simulink model "QD2_DroneStack_MPC"  (R2023a)
settings: Solver=ode1  StartTime=0.0  StopTime=inf  FixedStep=1/1000  RelTol=1e-3  EnableMultiTasking=on
InitFcn:
  | % QD2_DroneStack_MPC: rutas de la librería qd2_* y del mapeo de motores
  | qd2_d = fileparts(get_param(bdroot, 'FileName'));
  | for qd2_k = 1:4
  |     if exist(fullfile(qd2_d, 'lib', 'qd2_params.m'), 'file'), break; end
  |     qd2_d = fileparts(qd2_d);
  | end
  | addpath(fullfile(qd2_d, 'lib'));
  | addpath(fullfile(qd2_d, 'equipo2_original'));
  | clear qd2_d qd2_k
  | Motor_Mapping_7_Inch
model workspace (MAT data in the model file):
  target_system = 1
undefined symbols (not defined in the file): _Commander, _QDrone2, _Stabilizer, datetime, HIL, KT, lf, log_, m, Motor_Matrix, n, qc_get_step_size, s, saved_data
libraries: quarc_library x94, simulink x27, simulink_extras x9
(part 4 of 5)

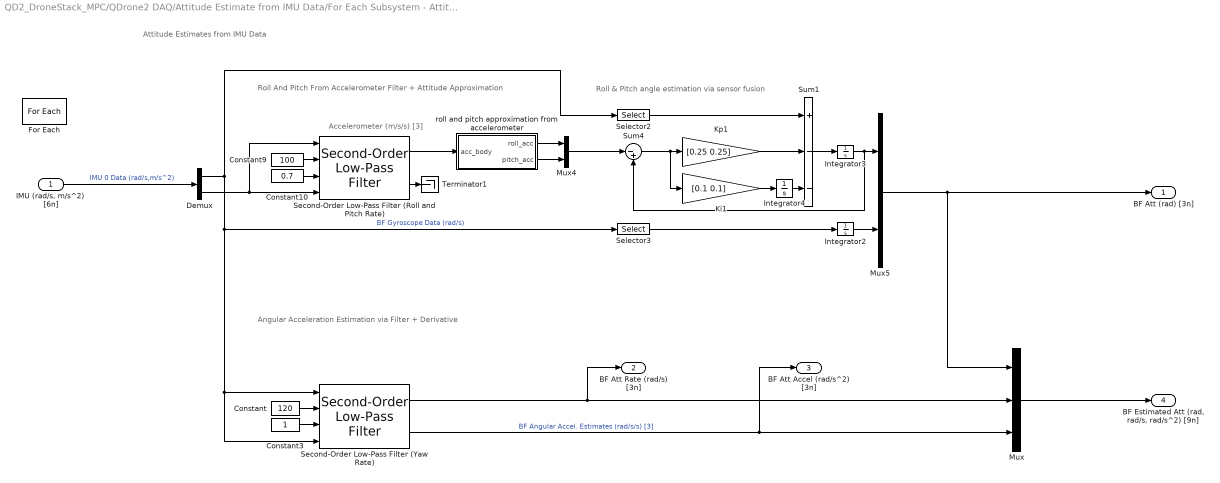
== system QD2_DroneStack_MPC/QDrone2 DAQ/Attitude Estimate from IMU Data/For Each Subsystem - Attitutde Estimates ==
  note: Attitude Estimates from IMU Data
  note: Accelerometer (m/s/s) [3]
  note: Roll And Pitch From Accelerometer Filter + Attitude Approximation
  note: Roll & Pitch angle estimation via sensor fusion
  note: Angular Acceleration Estimation via Filter + Derivative
  "IMU (rad/s, m/s^2) [6n]" : Inport  Partition=on  PartitionDimension=1  PartitionWidth=6  PartitionOffset=0
  Constant : Constant  Value=120
  Constant10 : Constant  Value=0.7
  Constant3 : Constant
  Constant9 : Constant  Value=100
  Demux : Demux  Outputs=[3,3]
  For Each : ForEach  DisableCoverage=on
  Integrator2 : Integrator
  Integrator3 : Integrator
  Integrator4 : Integrator
  Ki1 : Gain  Gain=[0.1 0.1]
  Kp1 : Gain  Gain=[0.25 0.25]
  Mux : Mux  Inputs=3
  Mux4 : Mux  Inputs=2
  Mux5 : Mux  Inputs=2
  Second-Order Low-Pass Filter (Roll and Pitch Rate) : quarc_library/Continuous/Second-Order Low-Pass Filter  params_source=External (input ports)  input_width=200  input_zeta=1  input_init=0
  Second-Order Low-Pass Filter (Yaw Rate) : quarc_library/Continuous/Second-Order Low-Pass Filter  params_source=External (input ports)  input_width=200  input_zeta=1  input_init=0
  Selector2 : Selector  InputPortWidth=3  IndexOptions=Index vector (dialog)  Indices=[1,2]  OutputSizes=1
  Selector3 : Selector  InputPortWidth=3  IndexOptions=Index vector (dialog)  Indices=[3]  OutputSizes=1
  Sum1 : Sum  Inputs=+--
  Sum4 : Sum  Inputs=|-+
  Terminator1 : Terminator
  roll and pitch approximation from accelerometer : MATLAB Function  TreatAsAtomicUnit=on
  BF Att (rad) [3n] : Outport  ConcatenationDimension=1
  BF Att Rate (rad/s) [3n] : Outport  Port=2  ConcatenationDimension=1
  BF Att Accel (rad/s^2) [3n] : Outport  Port=3  ConcatenationDimension=1
  "BF Estimated Att (rad, rad/s, rad/s^2) [9n] " : Outport  Port=4  ConcatenationDimension=1
  wires:
  roll and pitch approximation from accelerometer/2(pitch_acc) -> Mux4/2
  Constant9/1 -> Second-Order Low-Pass Filter (Roll and Pitch Rate)/2
  Second-Order Low-Pass Filter (Roll and Pitch Rate)/1 -> roll and pitch approximation from accelerometer/1(acc_body)
  "IMU (rad/s, m/s^2) [6n]"/1 -> Demux/1  "IMU 0 Data (rad/s,m/s^2)"
  Constant10/1 -> Second-Order Low-Pass Filter (Roll and Pitch Rate)/3
  Demux/2 -> Second-Order Low-Pass Filter (Roll and Pitch Rate)/4, Second-Order Low-Pass Filter (Roll and Pitch Rate)/1
  Second-Order Low-Pass Filter (Roll and Pitch Rate)/2 -> Terminator1/1
  Selector3/1 -> Integrator2/1
  Integrator2/1 -> Mux5/2
  Integrator4/1 -> Sum1/3
  Kp1/1 -> Sum1/2
  Selector2/1 -> Sum1/1
  Integrator3/1 -> Sum4/2, Mux5/1
  Mux5/1 -> BF Att (rad) [3n]/1, Mux/1
  Sum4/1 -> Ki1/1, Kp1/1
  Sum1/1 -> Integrator3/1
  Ki1/1 -> Integrator4/1
  roll and pitch approximation from accelerometer/1(roll_acc) -> Mux4/1
  Mux4/1 -> Sum4/1
  Constant3/1 -> Second-Order Low-Pass Filter (Yaw Rate)/3
  Demux/1 -> Second-Order Low-Pass Filter (Yaw Rate)/4, Second-Order Low-Pass Filter (Yaw Rate)/1, Selector3/1, Selector2/1  "BF Gyroscope Data (rad/s)"
  Constant/1 -> Second-Order Low-Pass Filter (Yaw Rate)/2
  Second-Order Low-Pass Filter (Yaw Rate)/1 -> Mux/2, BF Att Rate (rad/s) [3n]/1
  Second-Order Low-Pass Filter (Yaw Rate)/2 -> BF Att Accel (rad/s^2) [3n]/1, Mux/3  "BF Angular Accel. Estimates (rad/s/s) [3]"
  Mux/1 -> "BF Estimated Att (rad, rad/s, rad/s^2) [9n] "/1

== system QD2_DroneStack_MPC/QDrone2 DAQ/Check Battery level/Triggered Subsystem ==
  Trigger : TriggerPort  VariantControl=(inherit)
  Constant : Constant
  Out1 : Outport  InitialOutput=[0]
  wires:
  Constant/1 -> Out1/1

== system QD2_DroneStack_MPC/QDrone2 DAQ/Sensor Failure Monitoring - IMU0/Sensor Failure (Accelerometer) ==
  note: Check for flat-line ZERO Accelerometer data (no data)
  Sensor Input : Inport
  Clock : Clock
  Compare To Constant : simulink/Logic and Bit Operations/Compare To Constant  relop=>=  const=1  OutDataTypeStr=boolean
  Demux1 : Demux  Outputs=3
  Logical Operator : Logic  Operator=OR  Inputs=3  AllPortsSameDT=off  OutDataTypeStr=boolean
  Logical Operator1 : Logic  AllPortsSameDT=off  OutDataTypeStr=boolean
  Terminator1 : Terminator
  Terminator3 : Terminator
  Terminator4 : Terminator
  Threshold : quarc_library/Discontinuities/Threshold  operator===  param_src=Specify via dialog  threshold=0  duration=1
      settings: SourceProductName=QUARC Targets
  Threshold1 : quarc_library/Discontinuities/Threshold  operator===  param_src=Specify via dialog  threshold=0  duration=1
      settings: SourceProductName=QUARC Targets
  Threshold2 : quarc_library/Discontinuities/Threshold  operator===  param_src=Specify via dialog  threshold=0  duration=1
      settings: SourceProductName=QUARC Targets
  Sensor Fault : Outport  VectorParamsAs1DForOutWhenUnconnected=off
  wires:
  Clock/1 -> Compare To Constant/1
  Threshold/1 -> Logical Operator/1
  Threshold1/1 -> Logical Operator/2
  Compare To Constant/1 -> Logical Operator1/1
  Logical Operator1/1 -> Sensor Fault/1
  Sensor Input/1 -> Demux1/1
  Threshold2/2 -> Terminator4/1
  Threshold2/1 -> Logical Operator/3
  Demux1/1 -> Threshold/1
  Demux1/3 -> Threshold2/1
  Demux1/2 -> Threshold1/1
  Logical Operator/1 -> Logical Operator1/2
  Threshold1/2 -> Terminator3/1
  Threshold/2 -> Terminator1/1

== system QD2_DroneStack_MPC/QDrone2 DAQ/Sensor Failure Monitoring - IMU0/Sensor Failure (Gyroscope) ==
  note: Check for flat-line ZERO Gyro data (no data)
  Sensor Input : Inport
  Clock : Clock
  Compare To Constant : simulink/Logic and Bit Operations/Compare To Constant  relop=>=  const=1  OutDataTypeStr=boolean
  Demux1 : Demux  Outputs=3
  Logical Operator : Logic  Operator=OR  Inputs=3  AllPortsSameDT=off  OutDataTypeStr=boolean
  Logical Operator1 : Logic  AllPortsSameDT=off  OutDataTypeStr=boolean
  Terminator1 : Terminator
  Terminator3 : Terminator
  Terminator4 : Terminator
  Threshold : quarc_library/Discontinuities/Threshold  operator===  param_src=Specify via dialog  threshold=0  duration=1
      settings: SourceProductName=QUARC Targets
  Threshold1 : quarc_library/Discontinuities/Threshold  operator===  param_src=Specify via dialog  threshold=0  duration=1
      settings: SourceProductName=QUARC Targets
  Threshold2 : quarc_library/Discontinuities/Threshold  operator===  param_src=Specify via dialog  threshold=0  duration=1
      settings: SourceProductName=QUARC Targets
  Sensor Fault : Outport  VectorParamsAs1DForOutWhenUnconnected=off
  wires:
  Threshold/2 -> Terminator1/1
  Threshold1/2 -> Terminator3/1
  Logical Operator/1 -> Logical Operator1/2
  Demux1/2 -> Threshold1/1
  Demux1/3 -> Threshold2/1
  Demux1/1 -> Threshold/1
  Threshold2/1 -> Logical Operator/3
  Threshold2/2 -> Terminator4/1
  Sensor Input/1 -> Demux1/1
  Logical Operator1/1 -> Sensor Fault/1
  Compare To Constant/1 -> Logical Operator1/1
  Threshold1/1 -> Logical Operator/2
  Threshold/1 -> Logical Operator/1
  Clock/1 -> Compare To Constant/1

== system QD2_DroneStack_MPC/QDrone2 DAQ/Sensor Failure Monitoring - IMU1/Sensor Failure (Accelerometer) ==
  note: Check for flat-line ZERO Accelerometer data (no data)
  Sensor Input : Inport
  Clock : Clock
  Compare To Constant : simulink/Logic and Bit Operations/Compare To Constant  relop=>=  const=1  OutDataTypeStr=boolean
  Demux1 : Demux  Outputs=3
  Logical Operator : Logic  Operator=OR  Inputs=3  AllPortsSameDT=off  OutDataTypeStr=boolean
  Logical Operator1 : Logic  AllPortsSameDT=off  OutDataTypeStr=boolean
  Terminator1 : Terminator
  Terminator3 : Terminator
  Terminator4 : Terminator
  Threshold : quarc_library/Discontinuities/Threshold  operator===  param_src=Specify via dialog  threshold=0  duration=1
      settings: SourceProductName=QUARC Targets
  Threshold1 : quarc_library/Discontinuities/Threshold  operator===  param_src=Specify via dialog  threshold=0  duration=1
      settings: SourceProductName=QUARC Targets
  Threshold2 : quarc_library/Discontinuities/Threshold  operator===  param_src=Specify via dialog  threshold=0  duration=1
      settings: SourceProductName=QUARC Targets
  Sensor Fault : Outport  VectorParamsAs1DForOutWhenUnconnected=off
  wires:
  Threshold/2 -> Terminator1/1
  Threshold1/2 -> Terminator3/1
  Logical Operator/1 -> Logical Operator1/2
  Demux1/2 -> Threshold1/1
  Demux1/3 -> Threshold2/1
  Demux1/1 -> Threshold/1
  Threshold2/1 -> Logical Operator/3
  Threshold2/2 -> Terminator4/1
  Sensor Input/1 -> Demux1/1
  Logical Operator1/1 -> Sensor Fault/1
  Compare To Constant/1 -> Logical Operator1/1
  Threshold1/1 -> Logical Operator/2
  Threshold/1 -> Logical Operator/1
  Clock/1 -> Compare To Constant/1

== system QD2_DroneStack_MPC/QDrone2 DAQ/Sensor Failure Monitoring - IMU1/Sensor Failure (Gyroscope) ==
  note: Check for flat-line ZERO Gyro data (no data)
  Sensor Input : Inport
  Clock : Clock
  Compare To Constant : simulink/Logic and Bit Operations/Compare To Constant  relop=>=  const=1  OutDataTypeStr=boolean
  Demux1 : Demux  Outputs=3
  Logical Operator : Logic  Operator=OR  Inputs=3  AllPortsSameDT=off  OutDataTypeStr=boolean
  Logical Operator1 : Logic  AllPortsSameDT=off  OutDataTypeStr=boolean
  Terminator1 : Terminator
  Terminator3 : Terminator
  Terminator4 : Terminator
  Threshold : quarc_library/Discontinuities/Threshold  operator===  param_src=Specify via dialog  threshold=0  duration=1
      settings: SourceProductName=QUARC Targets
  Threshold1 : quarc_library/Discontinuities/Threshold  operator===  param_src=Specify via dialog  threshold=0  duration=1
      settings: SourceProductName=QUARC Targets
  Threshold2 : quarc_library/Discontinuities/Threshold  operator===  param_src=Specify via dialog  threshold=0  duration=1
      settings: SourceProductName=QUARC Targets
  Sensor Fault : Outport  VectorParamsAs1DForOutWhenUnconnected=off
  wires:
  Clock/1 -> Compare To Constant/1
  Threshold/1 -> Logical Operator/1
  Threshold1/1 -> Logical Operator/2
  Compare To Constant/1 -> Logical Operator1/1
  Logical Operator1/1 -> Sensor Fault/1
  Sensor Input/1 -> Demux1/1
  Threshold2/2 -> Terminator4/1
  Threshold2/1 -> Logical Operator/3
  Demux1/1 -> Threshold/1
  Demux1/3 -> Threshold2/1
  Demux1/2 -> Threshold1/1
  Logical Operator/1 -> Logical Operator1/2
  Threshold1/2 -> Terminator3/1
  Threshold/2 -> Terminator1/1

== system QD2_DroneStack_MPC/QDrone2 DAQ/Subsystem1/Maintain previous value4 ==
  Value in : Inport
  Memory : Memory
  Switch : Switch  Criteria=u2 ~= 0  SaturateOnIntegerOverflow=off  InputSameDT=off
  Non 0 values : Outport
  wires:
  Value in/1 -> Switch/1, Switch/2
  Switch/1 -> Memory/1, Non 0 values/1
  Memory/1 -> Switch/3

== system QD2_DroneStack_MPC/COMMANDER (ANGLE MODE)/STATE MACHINE SIGNALS/Generate Extra Messages for Console/Boolean Edge-Based Triggered Print ==
  Signal Enable : Inport  Partition=on  PartitionDimension=1  PartitionWidth=1  PartitionOffset=0
  Message : Inport  Port=2  Partition=on  PartitionDimension=2  PartitionWidth=1  PartitionOffset=0
  time (s) : Inport  Port=3
  For Each : ForEach  DisableCoverage=on
  Triggered Subsystem1 : Subsystem  TreatAsAtomicUnit=on
  Out1 : Outport  ConcatenationDimension=1
  wires:
  time (s)/1 -> Triggered Subsystem1/1(Time (s))
  Message/1 -> Triggered Subsystem1/2(Message)
  Signal Enable/1 -> Out1/1, Triggered Subsystem1/Trigger

== system QD2_DroneStack_MPC/COMMANDER (ANGLE MODE)/STATE MACHINE SIGNALS/Generate State Messages for Console/Triggered Subsystem ==
  Value : Inport
  Time (s) : Inport  Port=2
  Message : Inport  Port=3
  Trigger : TriggerPort  VariantControl=(inherit)
  Data Type Conversion : DataTypeConversion  OutDataTypeStr=uint8  SaturateOnIntegerOverflow=off  RndMeth=Floor
  Print : quarc_library/User Interface/Standard I//O/Print  format_string="[ %lf ] (s): State %u  => %s \\n"  max_code_units=512  optimization=Minimizing latency  sample_time=-1  active=off
      settings: SourceProductName=QUARC Targets
  Terminator : Terminator
  Terminator1 : Terminator
  wires:
  Time (s)/1 -> Print/1
  Message/1 -> Print/3
  Print/2 -> Terminator/1
  Print/1 -> Terminator1/1
  Value/1 -> Data Type Conversion/1
  Data Type Conversion/1 -> Print/2

== system QD2_DroneStack_MPC/COMMANDER (ANGLE MODE)/STATE MACHINE SIGNALS/Generate Warning Messages for Console/Boolean Value-Based Triggered Print ==
  Signal Enable : Inport  Partition=on  PartitionDimension=1  PartitionWidth=1  PartitionOffset=0
  Message : Inport  Port=2  Partition=on  PartitionDimension=2  PartitionWidth=1  PartitionOffset=0
  time (s) : Inport  Port=3
  For Each : ForEach  DisableCoverage=on
  Triggered Subsystem : Subsystem  TreatAsAtomicUnit=on
  Out1 : Outport  ConcatenationDimension=1
  wires:
  time (s)/1 -> Triggered Subsystem/1(Time (s))
  Message/1 -> Triggered Subsystem/2(Message)
  Signal Enable/1 -> Triggered Subsystem/Trigger, Out1/1

== system QD2_DroneStack_MPC/COMMANDER (ANGLE MODE)/STATE MACHINE SIGNALS/Generate Extra Messages for Console/Boolean Edge-Based Triggered Print/Triggered Subsystem1 ==
  Time (s) : Inport
  Message : Inport  Port=2
  Trigger : TriggerPort  TriggerType=falling  VariantControl=(inherit)
  Print : quarc_library/User Interface/Standard I//O/Print  format_string=[ %lf ] (s): %s !\n  max_code_units=512  optimization=Minimizing latency  sample_time=-1  active=off
      settings: SourceProductName=QUARC Targets
  Terminator : Terminator
  Terminator1 : Terminator
  wires:
  Time (s)/1 -> Print/1
  Message/1 -> Print/2
  Print/2 -> Terminator/1
  Print/1 -> Terminator1/1

== system QD2_DroneStack_MPC/COMMANDER (ANGLE MODE)/STATE MACHINE SIGNALS/Generate Warning Messages for Console/Boolean Value-Based Triggered Print/Triggered Subsystem ==
  Time (s) : Inport
  Message : Inport  Port=2
  Trigger : TriggerPort  VariantControl=(inherit)
  Print : quarc_library/User Interface/Standard I//O/Print  format_string=[ %lf ] (s): %s\n  max_code_units=512  optimization=Minimizing latency  sample_time=-1  active=off
      settings: SourceProductName=QUARC Targets
  Terminator : Terminator
  Terminator1 : Terminator
  wires:
  Print/1 -> Terminator1/1
  Print/2 -> Terminator/1
  Message/1 -> Print/2
  Time (s)/1 -> Print/1

== matlab function QD2_DroneStack_MPC/HORIZON FRAME CONVERSION AND ESTIMATION/Pose Switchbox/MATLAB Function2 ==
  data: sigmoid_type input; enable output; height_des input; slow_lim input; fast_lim input; height_cur input; height_vel input; height_ref output; max_height_vel output; max_height_accel output
function [enable, height_ref, max_height_vel, max_height_accel] = fcn(sigmoid_type, height_des, slow_lim, fast_lim, height_cur, height_vel)

% Note: Some of the cases below are identical. However, they are separated out 
% based on the states of the state machine for ease of modification in the future. 
% For example, states 4 and 5 are identical. However, if the user wants different 
% signmoid behaviour when taking off than when landing, these cases may not be the same. 

enable = 0;
height_ref = 0;
max_height_vel = 0;
max_height_accel = 0;

switch sigmoid_type
    case 1 % This is for the IDLE, ARM, E_ABORT, E_STOP and DISABLE states of the FSM
        enable = 0;
        height_ref = 0;
        max_height_vel = 0;
        max_height_accel = 0;

    case 2 % This is for the TAKEOFF THROTTLE state of the FSM
        enable = 0;
        height_ref = 0;
        max_height_vel = 0;
        max_height_accel = 0;

    case 3 % This is for the FLIGHT state of the FSM 
        enable = 1;
        height_ref = height_des;
        max_height_vel = fast_lim(1);
        max_height_accel = fast_lim(2);

    case 4 % This is for the TAKEOFF HEIGHT state of the FSM
        enable = 1;
        height_ref = height_des;
        if (height_vel < 0)||(abs(height_cur - height_des) <= 0.1)||(height_des <= height_cur)
            max_height_vel = fast_lim(1);
            max_height_accel = fast_lim(2);
        else    
            max_height_vel = slow_lim(1);
            max_height_accel = slow_lim(2);
        end
    case 5 % This is for the AUTOLAND state of the FSM
        enable = 1;
        height_ref = 0;
        if height_vel >= 0
            max_height_vel = fast_lim(1);
            max_height_accel = fast_lim(2);        
        else
            max_height_vel = slow_lim(1);
            max_height_accel = slow_lim(2);
        end
        
end

== matlab function QD2_DroneStack_MPC/HORIZON FRAME CONVERSION AND ESTIMATION/Pose Switchbox/MATLAB Function4 ==
  data: sigmoid_type input; enable output; yaw_des input; slow_lim input; fast_lim input; yaw_cur input; yaw_ref output; max_yaw_vel output; max_yaw_accel output; yaw_vel input
function [enable, yaw_ref, max_yaw_vel, max_yaw_accel] = fcn(sigmoid_type, yaw_des, slow_lim, fast_lim, yaw_cur, yaw_vel)

% Note: Some of the cases below are identical. However, they are separated out 
% based on the states of the state machine for ease of modification in the future. 
% For example, states 4 and 5 are identical. However, if the user wants different 
% signmoid behaviour when taking off than when landing, these cases may not be the same. 

enable = 0;
yaw_ref = 0;
max_yaw_vel = 0;
max_yaw_accel = 0;

switch sigmoid_type
    case 1 % This is for the IDLE, ARM, E_ABORT, E_STOP and DISABLE states of the FSM
        enable = 0;
        yaw_ref = 0;
        max_yaw_vel = 0;
        max_yaw_accel = 0;
    case 2 % This is for the TAKEOFF THROTTLE state of the FSM
        enable = 1;
        yaw_ref = yaw_des;
        max_yaw_vel = slow_lim(1);
        max_yaw_accel = slow_lim(2);  
    case 3 % This is for the FLIGHT state of the FSM 
        enable = 1;
        yaw_ref = yaw_des;
        max_yaw_vel = fast_lim(1);
        max_yaw_accel = fast_lim(2);
    case 4 % This is for the TAKEOFF HEIGHT state of the FSM
        enable = 1;
        yaw_ref = yaw_des;
        if (yaw_vel < 0)||(yaw_des < yaw_cur)||(abs(yaw_cur-yaw_des)<=0.2)
            max_yaw_vel = fast_lim(1);
            max_yaw_accel = fast_lim(2);
        else    
            max_yaw_vel = slow_lim(1);
            max_yaw_accel = slow_lim(2);
        end
    case 5 % This is for the AUTOLAND state of the FSM
        enable = 1;
        yaw_ref = yaw_des;
        if (yaw_vel >= 0)
            max_yaw_vel = fast_lim(1);
            max_yaw_accel = fast_lim(2);
        else    
            max_yaw_vel = slow_lim(1);
            max_yaw_accel = slow_lim(2);
        end
end

== matlab function QD2_DroneStack_MPC/HORIZON FRAME CONVERSION AND ESTIMATION/Pose Switchbox/Signmoid Type ==
  data: FSM_state input; sigmoid_type output
function sigmoid_type  = sigmoid_type_position(FSM_state)

% QDrone: Position Switchbox
%
% Switching between different sigmoid types based on 
% which state the FSM is in.
%
% v3.0 - 4th October, 2018
%
% INPUTS:
% -------
% FSM_state = current state of the FSM------------------------------------------------------- (#)         [1]
% 
% OUTPUTS:
% --------
% sigmoid_type = an integer whose state determines how the commands/measurements are transformed-- (#)         [1]

% Sigmoid_type = 1; This is for the IDLE, ARM, E_ABORT, E_STOP and DISABLE states of the FSM
% Sigmoid_type = 2; This is for the TAKEOFF THROTTLE state of the FSM
% Sigmoid_type = 3; This is for the FLIGHT state of the FSM
% Sigmoid_type = 4; This is for the TAKEOFF HEIGHT state of the FSM
% Sigmoid_type = 5; This is for the AUTOLAND state of the FSM

sigmoid_type = 0;

switch FSM_state
    case 1 % IDLE STATE
        sigmoid_type = 1;
    case 2 % ARM STATE
        sigmoid_type = 1;
    case 3 % TAKEOFF THROTTLE STATE
        sigmoid_type = 2;
    case 4 % TAKEOFF HEIGHT STATE
        sigmoid_type = 4;
    case 5 % FLIGHT STATE
        sigmoid_type = 3;
    case 6 % AUTOLAND STATE
        sigmoid_type = 5;
    case 7 % EMERGENCY STOP STATE
        sigmoid_type = 1;
    case 8 % EMERGENCY ABORT STATE
        sigmoid_type = 1;
    case 9 % DISABLE STATE
        sigmoid_type = 1;
end

== matlab function QD2_DroneStack_MPC/COMMANDER (ANGLE MODE)/THROTTLE SWITCHBOX /Hover Throttle Sigmoid Parameters ==
  data: sigmoid_type input; enable output; trim_throttle input; takeoff_lim input; land_lim input; throttle_vel input; throttle_ref output; max_throttle_vel output; max_throttle_accel output
function [enable, throttle_ref, max_throttle_vel, max_throttle_accel] = fcn(sigmoid_type, trim_throttle, takeoff_lim, land_lim, throttle_vel)

% Note: Some of the cases below are identical. However, they are separated out 
% based on the states of the state machine for ease of modification in the future. 
% For example, states 4 and 5 are identical. However, if the user wants different 
% signmoid behaviour when taking off than when landing, these cases may not be the same. 

enable = 0;
throttle_ref = 0;
max_throttle_vel = 0;
max_throttle_accel = 0;

switch sigmoid_type
    case 1 % sigmoid = 1 - Command 0 throttle
        % This is for the IDLE, ARM, E_ABORT, and DISABLE states of the FSM
        enable = 0;
        throttle_ref = 0;
        max_throttle_vel = 0;
        max_throttle_accel = 0;

    case 2 % sigmoid = 2 - Sigmoid throttle up from 0 to the trim value
        % This is for the TAKEOFF THROTTLE state of the FSM
        enable = 1;
        throttle_ref = trim_throttle;
        max_throttle_vel = takeoff_lim(1);
        max_throttle_accel = takeoff_lim(2);

    case 3 % sigmoid = 3 - Pass controller throttle straight through + trim value.
        % This is for the TAKEOFF HEIGHT and FLIGHT state of the FSM
        enable = 1;
        throttle_ref = trim_throttle;
        max_throttle_vel = takeoff_lim(1);
        max_throttle_accel = takeoff_lim(2);

    case 4 % sigmoid = 4 - Ignore controller throttle. Sigmoid it down to 0.
        % This is for the E_Landing state of the FSM
        enable = 1;
        throttle_ref = 0;
        if throttle_vel > 0
            max_throttle_vel = takeoff_lim(1);
            max_throttle_accel = takeoff_lim(2);
        else
            max_throttle_vel = land_lim(1);
            max_throttle_accel = land_lim(2);
        end
        
    case 5 % sigmoid = 5 - Pass controller throttle straight through + trim value.
        % This is for the AUTOLAND state of the FSM
        enable = 1;
        throttle_ref = trim_throttle;
        max_throttle_vel = takeoff_lim(1);
        max_throttle_accel = takeoff_lim(2);

end

== matlab function QD2_DroneStack_MPC/COMMANDER (ANGLE MODE)/STATE MACHINE LOGIC ==
  data: E_Abort output; isArm output; pt_ARM_to_TAKEOFF_THROTTLE output; pt_TAKE_OFF_HEIGHT_TO_AUTOLAND output; pt_FLIGHT_TO_AUTOLAND output; current_state input; initializing input; Tracking_Issue input; Communication_Issue input; low_battery input; trigger_1 input; trigger_2 input; E_abort input; joystick_issue input; net_throttle_at_trim input; net_throttle_close_to_zero input; ctrl_throttle_close_to_zero input; take_off_successful input; flying_too_low input; flying_too_high input; close_to_ground input; pt_TAKEOFF_THROTTLE_TO_TAKEOFF_HEIGHT output; pt_TAKE_OFF_HEIGHT_TO_FLIGHT output; pt_AUTOLAND_TO_DISABLE output; pt_EMERGENCY_STOP_TO_DISABLE output; pt_EMERGENCY_ABORT_TO_DISABLE output; Error output; stop_model output; sensor_failed input
function [E_Abort, isArm, pt_ARM_to_TAKEOFF_THROTTLE, pt_TAKE_OFF_HEIGHT_TO_AUTOLAND, pt_FLIGHT_TO_AUTOLAND, pt_TAKEOFF_THROTTLE_TO_TAKEOFF_HEIGHT, pt_TAKE_OFF_HEIGHT_TO_FLIGHT, pt_AUTOLAND_TO_DISABLE, pt_EMERGENCY_STOP_TO_DISABLE, pt_EMERGENCY_ABORT_TO_DISABLE, Error, stop_model]...
    = SM_logic(current_state, initializing, Tracking_Issue, Communication_Issue, low_battery, trigger_1, trigger_2, E_abort, joystick_issue,...
    net_throttle_at_trim, net_throttle_close_to_zero, ctrl_throttle_close_to_zero, take_off_successful, flying_too_low, flying_too_high, close_to_ground, sensor_failed)

% Programmatic Logic Block
%
% Logic for the FSM is generated here based on a variety of signals.
% Mostly, logic to programmatically trigger the transition to either a 
% natural next state, or an Error state, is generated here.
%
% Last modified: March, 2020
%
% INPUTS:
% -------
% current_state = previous state of the FSM-------------------------------------------------- (#)         [1]
% initializing = signal representing that the system is initializing (first 5s + buffer)- - - (bool)      [1]
% comm = communication signal representing MAVLINK connection-------------------------------- (bool)      [1]
% peripheral = signal representing joystick and optitrack connection- - - - - - - - - - - - - (bool)      [2]
% low_battery = signal representing low battery---------------------------------------------- (bool)      [1]
% trigger_1 = trigger representing ARM/DISARM - - - - - - - - - - - - - - - - - - - - - - - - (bool)      [1]
% trigger_2 = trigger representing TAKEOFF/AUTOLAND------------------------------------------ (bool)      [1]
% motors_not_spinning = signal representing the motors not spinning - - - - - - - - - - - - - (bool)      [1]
% net_throttle_at_trim = trim throttle for the application drone ---------------------------- (bool)      [1]
% net_throttle_close_to_zero = net throttle is close to zero in emergency stop mode - - - - - (bool)      [1]
% ctrl_throttle_close_to_zero = ctrl throttle is close to zero in emergency stop mode - - - - (bool)      [1]
% take_off_successful = signal representing whether drone has taken-off successfully -------- (bool)      [1]
% flying_too_low = signal representing whether the drone's height is below threshold and cmd- (bool)      [1]
% flying_too_high = signal representing whether the drone's height is above threshold-------- (bool)      [1]
% close_to_ground = signal representing whether the drone is close to the ground to autoland- (bool)      [1]
% 
% OUTPUTS:
% --------
% Error = Whether an Error is issued or not                                                             (bool)    [1]
% E_Abort = fed through for ease of understanding flow (see STATE MACHINE TRANSITION BLOCK)             (bool)    [1]
% isArm = programmatic transition state                                                                 (bool)    [1]
% takeoff = fed through for ease of understanding flow (see STATE MACHINE TRANSITION BLOCK)             (bool)    [1]
% pt_ARM_to_TAKEOFF_THROTTLE = programmatic transition state BEGIN_STATE_TO_FINAL_STATE                 (bool)    [1]
% pt_TAKEOFF_THROTTLE_TO_TAKEOFF_HEIGHT = programmatic transition state BEGIN_STATE_TO_FINAL_STATE      (bool)    [1]
% pt_TAKE_OFF_HEIGHT_TO_AUTOLAND = programmatic transition state BEGIN_STATE_TO_FINAL_STATE             (bool)    [1]
% pt_TAKEOFF_THROTTLE_TO_TAKEOFF_HEIGHT = programmatic transition state BEGIN_STATE_TO_FINAL_STATE      (bool)    [1]
% pt_TAKE_OFF_HEIGHT_TO_FLIGHT = programmatic transition state BEGIN_STATE_TO_FINAL_STATE               (bool)    [1]
% pt_AUTOLAND_TO_DISABLE = programmatic transition state BEGIN_STATE_TO_FINAL_STATE                     (bool)    [1]
% pt_EMERGENCY_STOP_TO_DISABLE = programmatic transition state BEGIN_STATE_TO_FINAL_STATE               (bool)    [1]
% pt_EMERGENCY_ABORT_TO_DISABLE = programmatic transition state BEGIN_STATE_TO_FINAL_STATE              (bool)    [1]
% stop_model = STOP THE MODEL AFTER                                                                     (bool)    [1]

Error = 0;
E_Abort = E_abort;
isArm = false;
pt_ARM_to_TAKEOFF_THROTTLE = false;
pt_TAKEOFF_THROTTLE_TO_TAKEOFF_HEIGHT = false;
pt_TAKE_OFF_HEIGHT_TO_AUTOLAND = false;
pt_TAKE_OFF_HEIGHT_TO_FLIGHT = false;
pt_FLIGHT_TO_AUTOLAND = false;
pt_AUTOLAND_TO_DISABLE = false;
pt_EMERGENCY_STOP_TO_DISABLE = false;
pt_EMERGENCY_ABORT_TO_DISABLE = false;
stop_model = 0;

switch current_state
    %---------------------------------------------------------------------%
    case 1 % IDLE STATE
        if (Communication_Issue)||...          % Communication issue
           (joystick_issue)||...               % joystick issue
           (Tracking_Issue)||...               % optitrack issue
           (low_battery)||...                  % low batter  
           (sensor_failed)||...                % if sensor (IMU) failure is detected on drone stabilizer    
           ((trigger_1)&&(initializing))||...  % armed while initializing
           (trigger_2)||...                    % tried to takeoff while initializing
           (~ctrl_throttle_close_to_zero)      % if throttle isn't at zero, don't arm
           %----------------------------------------%
            Error = 1;
        elseif trigger_1 % user arms
            isArm = true;
        end
    %---------------------------------------------------------------------%    
    case 2 % ARMED STATE
        isArm = trigger_1;
        if (Communication_Issue)||...          % Communication issue
           (joystick_issue)||...               % joystick issue
           (Tracking_Issue)||...               % optitrack issue
           (low_battery)||...                  % low battery
           (sensor_failed)||...                % if sensor (IMU) failure is detected on drone stabilizer
           (~ctrl_throttle_close_to_zero)      % if throttle isn't at zero, don't arm
           %----------------------------------------%
            Error = 1;
        elseif trigger_1 && trigger_2
            pt_ARM_to_TAKEOFF_THROTTLE = true;
        end        
    %---------------------------------------------------------------------%
    case 3 % TAKEOFF_THROTTLE STATE
        if (Communication_Issue)||...     % Communication issue
           (joystick_issue)||...          % joystick issue
           (Tracking_Issue)||...          % optitrack issue           
           (low_battery)||...             % low battery
           (sensor_failed)||...           % if sensor (IMU) failure is detected on drone stabilizer
           (~trigger_1)||...              % user disarms
           (~trigger_2)||...              % user commands auto-land before drone starts taking off
           (~ctrl_throttle_close_to_zero) % if throttle isn't at zero, don't arm
           %----------------------------------------%
            Error = 1;
        elseif net_throttle_at_trim
            pt_TAKEOFF_THROTTLE_TO_TAKEOFF_HEIGHT = true;
        end
    %---------------------------------------------------------------------%
    case 4 % TAKEOFF_HEIGHT STATE
        if (Communication_Issue)||... % Communication issue
           (joystick_issue)||...      % joystick issue
           (Tracking_Issue)||...      % optitrack issue
           (sensor_failed)||...       % if sensor (IMU) failure is detected on drone stabilizer    
           (flying_too_low)||...      % current height is below safety threshold 
           (flying_too_high)||...     % flying above safety margin (w.r.t optitrack)
           (~trigger_1)               % user disarms
            %----------------------------------------%
            Error = 1;
        elseif (~trigger_2)||low_battery 
            pt_TAKE_OFF_HEIGHT_TO_AUTOLAND = true;
        elseif take_off_successful
            pt_TAKE_OFF_HEIGHT_TO_FLIGHT = true;
        end
    %---------------------------------------------------------------------%
    case 5 % FLIGHT STATE
        if (Communication_Issue)||...   % Communication issue
           (joystick_issue)||...        % joystick issue
           (Tracking_Issue)||...        % optitrack issue
           (sensor_failed)||...         % if sensor (IMU) failure is detected on drone stabilizer
           (flying_too_low)||...        % current height is below safety threshold  
           (flying_too_high)||...       % flying above safety margin (w.r.t optitrack)
           (~trigger_1)                 % user disarms
           %----------------------------------------%
            Error = 1;
        elseif (~trigger_2)||low_battery
            pt_FLIGHT_TO_AUTOLAND = true;
        end
    %---------------------------------------------------------------------%
    case 6 % AUTOLAND STATE
        if (Communication_Issue)||...  % Communication issue
           (joystick_issue)||...       % joystick issue
           (Tracking_Issue)||...       % optitrack issue
           (sensor_failed)||...        % if sensor (IMU) failure is detected on drone stabilizer
           (flying_too_high)||...      % flying above safety margin (w.r.t optitrack)    
           (~trigger_1)                % user disarms
           %----------------------------------------%
            Error = 1;
        elseif close_to_ground 
            pt_AUTOLAND_TO_DISABLE = true;
        end
    %---------------------------------------------------------------------%
    case 7 % EMERGENCY LAND STATE
        if net_throttle_close_to_zero 
            pt_EMERGENCY_STOP_TO_DISABLE = true;
        end
    %---------------------------------------------------------------------%
    case 8 % EMERGENCY ABORT STATE
        pt_EMERGENCY_ABORT_TO_DISABLE = true;
    %---------------------------------------------------------------------%
    case 9
        % Stop the model.
        stop_model = 1;
end

== matlab function QD2_DroneStack_MPC/Communication/PROTOCOL CHECK ==
  data: rcv input; rcv_ok output size=24
function rcv_ok = fcn(rcv)
%#codegen
% PROTOCOL CHECK (versión MPC, 24 doubles, ARQUITECTURA.md 3.2).
% Acepta la trama solo si: arm, takeoff, e-stop, joystick_issue,
% isTracking (índices 1-5) y mpc_mode (23) valen exactamente 0 o 1, el
% índice 24 vale 2 (etiqueta de protocolo MPC v1, la manda tierra) y el
% timestamp (16) es finito y >= 0. Si no, repite la última trama válida
% (el timestamp congelado dispara la detección de pérdida de enlace).
persistent ult
if isempty(ult)
    ult = zeros(24, 1);
end
ok = true;
idx = [1 2 3 4 5 23];
for k = 1:6
    v = double(rcv(idx(k)));
    if ~(v == 0 || v == 1)
        ok = false;
    end
end
v24 = double(rcv(24));
if ~(v24 == 2)
    ok = false;
end
ts = double(rcv(16));
if ~(isfinite(ts) && ts >= 0)
    ok = false;
end
if ok
    ult = double(rcv(:));
end
rcv_ok = ult;

== matlab function QD2_DroneStack_MPC/COMMANDER (ANGLE MODE)/STATE MACHINE TRANSITION ==
  data: current_state input; E_Abort input; isArm input; pt_ARM_to_TAKEOFF_THROTTLE input; pt_TAKE_OFF_HEIGHT_TO_AUTOLAND input; pt_FLIGHT_TO_AUTOLAND input; Next_state output; pt_TAKEOFF_THROTTLE_TO_TAKEOFF_HEIGHT input; pt_TAKE_OFF_HEIGHT_TO_FLIGHT input; pt_AUTOLAND_TO_DISABLE input; pt_EMERGENCY_STOP_TO_DISABLE input; pt_EMERGENCY_ABORT_TO_DISABLE input; Error input
function Next_state = SM_transition(current_state, E_Abort, isArm, pt_ARM_to_TAKEOFF_THROTTLE, pt_TAKE_OFF_HEIGHT_TO_AUTOLAND, pt_FLIGHT_TO_AUTOLAND, pt_TAKEOFF_THROTTLE_TO_TAKEOFF_HEIGHT, pt_TAKE_OFF_HEIGHT_TO_FLIGHT, pt_AUTOLAND_TO_DISABLE, pt_EMERGENCY_STOP_TO_DISABLE, pt_EMERGENCY_ABORT_TO_DISABLE, Error)

% Programmatic Transition Block
%
% FINITE STATE MACHINE (FSM) with 9 states as described below, transitioning based on the 
% values of the isArm, transition signals, Error, and E_Abort
%
% Last modified: March, 2020
%
% INPUTS:
% ------
% current_state = Current state of the FSM        (#)     [1]
% E_Abort                                         (bool)  [1]
% isArm                                           (bool)  [1]
% pt_ARM_TO_TAKEOFF_THROTTLE                      (bool)  [1]
% pt_TAKE_OFF_HEIGHT_TO_AUTOLAND                  (bool)  [1]
% pt_FLIGHT_TO_AUTOLAND                           (bool)  [1]
% pt_TAKEOFF_THROTTLE_TO_TAKEOFF_HEIGHT           (bool)  [1]
% pt_TAKE_OFF_HEIGHT_TO_FLIGHT                    (bool)  [1]
% pt_AUTOLAND_TO_DISABLE                          (bool)  [1]
% pt_EMERGENCY_STOP_TO_DISABLE                    (bool)  [1]
% pt_EMERGENCY_ABORT_TO_DISABLE                   (bool)  [1]
% Error                                           (bool)  [1]
%
% OUTPUT:
% -------
% Next_state = Next state of the FSM              (#)     [1]

Next_state = double(0);
switch current_state
%-------------------------------------------------------------------------%
    case 1 % IDLE STATE
        if E_Abort
            Next_state = 8; % GOTO EMERGENCY ABORT STATE
        elseif Error
            Next_state = 7; % GOTO EMERGENCY STOP STATE
        elseif isArm
            Next_state = 2; % GOTO ARMED STATE
        else
            Next_state = 1; % STAY IN IDLE STATE
        end
%-------------------------------------------------------------------------%
    case 2 % ARMED STATE
        if E_Abort
            Next_state = 8; % GOTO EMERGENCY ABORT STATE
        elseif Error
            Next_state = 7; % GOTO EMERGENCY STOP STATE
        elseif ~isArm
            Next_state = 1; % GOTO IDLE STATE
        elseif pt_ARM_to_TAKEOFF_THROTTLE
            Next_state = 3; % GOTO TAKEOFF_THROTTLE STATE 
        else
            Next_state = 2; % STAY IN ARMED STATE
        end
%-------------------------------------------------------------------------%
    case 3 % TAKEOFF_THROTTLE STATE
        if E_Abort
            Next_state = 8; % GOTO EMERGENCY ABORT STATE
        elseif Error
            Next_state = 7; % GOTO EMERGENCY STOP STATE
        elseif pt_TAKEOFF_THROTTLE_TO_TAKEOFF_HEIGHT
            Next_state = 4; % GOTO TAKEOFF_HEIGHT STATE
        else
            Next_state = 3; % STAY IN TAKEOFF_THROTTLE STATE
        end
%-------------------------------------------------------------------------%
    case 4 % TAKEOFF_HEIGHT STATE
        if E_Abort
            Next_state = 8; % GOTO EMERGENCY ABORT STATE
        elseif Error
            Next_state = 7; % GOTO EMERGENCY STOP STATE
        elseif pt_TAKE_OFF_HEIGHT_TO_AUTOLAND
            Next_state = 6;
        elseif pt_TAKE_OFF_HEIGHT_TO_FLIGHT
            Next_state = 5; % GOTO FLIGHT STATE
        else
            Next_state = 4; % STAY IN TAKEOFF_HEIGHT STATE
        end
%-------------------------------------------------------------------------%
    case 5 % FLIGHT STATE
        if E_Abort
            Next_state = 8; % GOTO EMERGENCY ABORT STATE
        elseif Error
            Next_state = 7; % GOTO EMERGENCY STOP STATE
        elseif pt_FLIGHT_TO_AUTOLAND
            Next_state = 6; % GOTO AUTO_LAND STATE
        else
            Next_state = 5; % STAY IN FLIGHT STATE
        end
%-------------------------------------------------------------------------%       
    case 6 % AUTO_LAND STATE
        if E_Abort
            Next_state = 8; % GOTO EMERGENCY ABORT STATE
        elseif Error
            Next_state = 7; % GOTO EMERGENCY STOP STATE
        elseif pt_AUTOLAND_TO_DISABLE
            Next_state = 9; % GOTO DISABLE STATE
        else
            Next_state = 6; % STAY IN AUTO_LAND STATE
        end
%-------------------------------------------------------------------------%
    case 7 % EMERGENCY STOP STATE
        if E_Abort
            Next_state = 8; % GOTO EMERGENCY ABORT STATE
        elseif pt_EMERGENCY_STOP_TO_DISABLE
            Next_state = 9; % GOTO DISABLE STATE
        else
            Next_state = 7; % STAY IN EMERGENCY STOP STATE
        end
%-------------------------------------------------------------------------%
    case 8 % EMERGENCY ABORT
        if pt_EMERGENCY_ABORT_TO_DISABLE
            Next_state = 9; % GOTO DISABLE STATE
        else 
            Next_state = 8; % STAY IN EMERGENCY ABORT STATE
        end
%-------------------------------------------------------------------------%    
    case 9 % DISABLE
        Next_state = 9; % Always stay in DISABLE state if you are here    
end

== matlab function QD2_DroneStack_MPC/COMMANDER (ANGLE MODE)/MPC POSITION CONTROLLER (50 Hz) ==
  data: u input; y output size=[7 1]
function y = fcn(u)
%#codegen
% MPC DE POSICIÓN A BORDO (50 Hz). Sustituye al PIV del COMMANDER cuando
% mpc_mode = 1 (índice 23 del paquete PC->dron, ARQUITECTURA.md 3.2).
% u (31x1): [IF Pose Info(8) = medida x y z yaw + deseada x y z yaw,
%            HF Pose Rate(4) = vx vy vz (horizon frame) + yaw rate,
%            Actitud estimada(9) = roll pitch yaw ..., datos MPC(8) =
%            otro dron x y z vx vy vz + mpc_mode + reservado,
%            estado FSM, empuje de hover (N)]
% y (7x1):  [comando (4) en el formato del PIV: T-trim, roll, pitch,
%            yaw_rate; usar_mpc (0/1); estado MPC; d_hat (m/s^2)]
% Estado MPC: 0 ok, 1 FISTA sin converger (se aplica igual), 2 entrada
% inválida (pasa el PIV), 3 inactivo (FSM fuera de 4-6), 4 PIV elegido
% (mpc_mode = 0, el MPC corre en sombra).
% Parámetros: qd2_params() se evalúa al COMPILAR (coder.const), así que el
% Jetson no corre la Riccati, expm ni los waypoints en la primera llamada.
P0 = coder.const(@feval, 'qd2_params');
persistent p mst activo_prev modo_prev masa_ok
if isempty(p)
    p = P0;
    mst = qd2_mpc_init(p);
    activo_prev = 0;
    modo_prev = 0;
    masa_ok = 0;
end
pose_if = u(1:8);
v_hf    = u(9:11);
att     = u(13:21);
otro    = u(22:27);
modo    = double(u(28) > 0.5);
fsm     = u(30);
T_hover = u(31);
% El MPC sigue al "Drone Weight" del modelo (mismo trim que el PIV). Si la
% masa difiere de qd2_params, se reconstruye UNA vez todo el modelo del MPC
% (trim, masa, matrices del eje z y cotas) con qd2_mpc_build. Solo se hace
% en tierra (FSM 1-2), nunca en vuelo.
if masa_ok < 0.5 && fsm <= 2 && isfinite(T_hover) && T_hover > 1
    masa_ok = 1;
    if abs(T_hover - p.T_trim) > 1e-3
        b.g = p.g;
        b.masa = T_hover/p.g;
        b.T_trim = T_hover;
        b.planta.tau_att = p.planta.tau_att;
        b.pid.Kp = p.pid.Kp;
        p.mpc = qd2_mpc_build(b);
        p.T_trim = T_hover;
        p.masa = b.masa;
        mst = qd2_mpc_init(p);
    end
end
activo = (fsm >= 4) && (fsm <= 6);
% Reinicio al entrar a TAKEOFF_HEIGHT (como el integrador del PIV) y al
% pasar de PIV a MPC en vuelo (el observador en sombra no vio el empuje real)
if activo && (activo_prev < 0.5 || (modo > 0.5 && modo_prev < 0.5))
    mst = qd2_mpc_init(p);
end
psi = pose_if(4);
c = cos(psi); s = sin(psi);
% velocidad del horizon frame al marco inercial (yaw medido)
x_est = [pose_if(1); pose_if(2); pose_if(3); ...
         c*v_hf(1) - s*v_hf(2); s*v_hf(1) + c*v_hf(2); v_hf(3); ...
         att(1); att(2); psi];
ref = [pose_if(5); pose_if(6); pose_if(7); pose_if(8)];
cmd = zeros(4,1);
usar = 0;
estado = 3;
d_hat = 0;
if activo
    [uu, mst, info] = qd2_mpc_position(x_est, ref, otro, p, mst);
    estado = uu(5);
    d_hat = info.d_hat;
    cmd = [uu(1) - p.T_trim; uu(2); uu(3); uu(4)];
    if estado < 1.5 && all(isfinite(cmd))
        if modo > 0.5
            usar = 1;
        else
            estado = 4;
        end
    else
        estado = 2;
        cmd = zeros(4,1);
    end
end
activo_prev = double(activo);
modo_prev = modo;
y = [cmd; usar; estado; d_hat];

== matlab function QD2_DroneStack_MPC/Communication/Detect Communication Loss/MATLAB Function ==
  settings: updateMethod=DISCRETE
  data: time input; stream_connection_loss output; state input; error input; ms_time input; data_loss output
function [stream_connection_loss , data_loss] = fcn(time, state, error, ms_time)

persistent ms_time_prev
    if isempty(ms_time_prev)
        ms_time_prev = 0;
    end

stream_connection_loss = 0;
data_loss = 0;
if time > 3
    if ((state ~= 2)&&(error < 0))
        % stream connection is not established correctly
        stream_connection_loss = 1;
    end

    if (ms_time == ms_time_prev)&&(ms_time > 0)
        % data is stale
        data_loss = 1;
    end
end

ms_time_prev = ms_time;

== matlab function QD2_DroneStack_MPC/QDrone2 DAQ/Force to percentage Mapping ==
  data: V_Bat_Act input; Motor_Forces input; Duty_Cycle output; KT input
function Duty_Cycle = fcn(V_Bat_Act,Motor_Forces,KT)

B = KT(2)^2-4*KT(1)*(KT(3)-Motor_Forces)

invalid_signal = B < 0
B(invalid_signal) = 0

% Ranges from 1000-2000
Volt_CMD_Theo = -0.5*KT(2)/KT(1)+ sqrt(B)/(2*KT(1));

Duty_Cycle = Volt_CMD_Theo/V_Bat_Act;

== matlab function QD2_DroneStack_MPC/QDrone2 DAQ/Attitude Estimate from IMU Data/For Each Subsystem - Attitutde Estimates/roll and pitch approximation from accelerometer ==
  data: roll_acc output; pitch_acc output; acc_body input
function [roll_acc, pitch_acc]   = fcn(acc_body)
%#eml
n = norm(acc_body,2);
if n>eps
    acc_body = acc_body/n; 
else
    acc_body = [0 0 1]';
end

roll_acc = atan2(acc_body(2),acc_body(3));
pitch_acc = atan2( -acc_body(1), acc_body(2)*sin(roll_acc)+acc_body(3)*cos(roll_acc));

== matlab function QD2_DroneStack_MPC/QDrone2 DAQ/Subsystem/MATLAB Function LED Color Assignment ==
  data: E_Stop input; Arm input; value output; low_battery input
function value = fcn(E_Stop, Arm, low_battery)

if low_battery == 1|| E_Stop ==1
    value = 1;
elseif Arm == 1 & E_Stop ==0
    value = 2;
elseif Arm == 0 && E_Stop == 0 
    value = 3;
else 
    value = 3;
end

== matlab function QD2_DroneStack_MPC/COMMANDER (ANGLE MODE)/THROTTLE SWITCHBOX /Throttle Switchbox ==
  data: FSM_state input; sigmoid output
function sigmoid  = application_drone_throttle_switchbox(FSM_state)

% Application Drone: Throttle Switchbox
%
% Logic for switching between throttle commands from the controller 
%
% v2.0 - 5th october, 2018
%
% INPUTS:
% -------
% FSM_state = current state of the FSM------------------------------------------------------- (#)         [1]
% 
% OUTPUTS:
% --------
% sigmoid = an integer whose state determines how the heights are transformed---------------- (#)         [1]
% sigmoid = 1 - Command 0 throttle
% sigmoid = 2 - Sigmoid throttle up from 0 to the trim value
% sigmoid = 3 - Pass controller throttle straight through + trim value.
% sigmoid = 4 - Ignore controller throttle. Sigmoid it down to 0.
% sigmoid = 5 - Pass controller throttle straight through + trim value.


sigmoid = 0;
switch FSM_state
    case 1 % IDLE STATE
        sigmoid = 1;
    case 2 % ARM STATE
        sigmoid = 1;
    case 3 % TAKEOFF THROTTLE STATE
        sigmoid = 2;
    case 4 % TAKEOFF HEIGHT STATE
        sigmoid = 3;
    case 5 % FLIGHT STATE
        sigmoid = 3;
    case 6 % AUTOLAND STATE
        sigmoid = 5;
    case 7 % EMERGENCY STOP STATE
        sigmoid = 4;
    case 8 % EMERGENCY ABORT STATE
        sigmoid = 1;
    case 9 % DISABLE STATE
        sigmoid = 1;
end

== matlab function QD2_DroneStack_MPC/QDrone2 DAQ/MotorCMD_FSM ==
  data: Arm_Signal input; E_Stop input; ESC_cmd output; Motor_State output; Model_Time input; Motor_State input
function [ESC_cmd,Motor_State]= fcn(Arm_Signal,E_Stop,Model_Time, Motor_State)

persistent state ESC_CMD 

%  Initialize motor state at the start of the model
if isempty(state)
    state = 2;
    ESC_CMD = zeros(1,4);
end 

% ESC Numbers w.r.t motor positions on QDrone: 
%         FRONT
%       4(3)       2(1)
% 
%       3(2)       1(0)
%          BACK  


% ============ Motor programing state machine ============ 

% State machine transitions: 

% Motor configuration state: 
if E_Stop == 0 && state ~= 9
    % Start with the motors in an idle state    
    if state == 2 && Model_Time > 0 && Model_Time <= 1  
        if Arm_Signal == 1
            % Error state, you started the model while the QDrone was armed
            state = 9;
        end 
           
    elseif state ==2  && Model_Time > 1 && Model_Time <= 2
        % Enter motor Low Frequency state:
        state = 1;
        
    elseif state ==1  && Model_Time > 2 && Model_Time <= 2.5
        % Set motor orientation
        state = 0;
        
    elseif state == 0 && Model_Time > 2.5    
        % Enter motor idle state: 
        state = 2; 

    elseif Motor_State ==2 && Arm_Signal == 1 
        % Enter arm state 
        state = 3;

    elseif Motor_State ==3 && Arm_Signal ==0 
        % Return to idle state 
        state = 2; 
    end 
    
elseif E_Stop ==1 
    % You've entered emergency state, disarm QDrone2!
    state = 9; 
end 


% State Machine commands: 
switch state 
    
    % ESC orientation set:
    case 0
        % for all drones
        ESC_CMD = [20,21,21,20];
        %for 1st R&D Drone 
        % ESC_CMD = [0,0,0,0];
    
    % Motor Low Frequency Beep:
    case 1
        ESC_CMD = [1,1,1,1];
    
    % Enter motor stop state: 
    case 2
        ESC_CMD = [0,0,0,0];
    
    % Motors in Arm State:
    case 3
        ESC_CMD = [48,48,48,48];
        
    % Same as state 2 but used as an Error State to stop motor cmd:
    case 9
        ESC_CMD = [0,0,0,0];
        
end 
    


Motor_State = state;
ESC_cmd = ESC_CMD;

Motor_State, ESC_cmd;
